simulink model "example_2"  (R2022b)
settings: Solver=VariableStepAuto  StartTime=0.0  StopTime=1  RelTol=1e-3
InitFcn:
  | %% Bộ biến đổi điện tử công suất
  | kb = 1;     % Hệ số khuếch đại khâu 1
  | f_switch = 53600; % (Hz) Tần số đóng cắt của bộ biến đổi
  | tb = 1/(2 * f_switch);   % Hằng số thời gian khâu 1
  | %% Động cơ
  | R = 0.6; % (Ohm) Điện trở động cơ
  | L = 1.5e-3; % (H) Điện cảm động cơ
  | k = 1/R; % Gain hàm truyền Plant
  | t = L/R; % Hằng số thời gian Plant
  | TL = 0.27; % Momen tải
  | ke = 0.064; % hằng số momen và hằng số sức điện động
  | J = 750e-3 * 10^(-4); % Momen quán tính động cơ
  | B = 0;
  | 
  | %% Bộ điều khiển
  | %omega_BW = 2 * pi * 1000;
  | omega_BW = 2*pi*f_switch/10;
  | Ti = t;
  | kp = R*Ti*omega_BW*sqrt(1 + (omega_BW*tb)^2)/kb;
  | ki = kp/Ti;
  | %Ts = 1e-5; % Thời gian trích mẫu
  | Ts = 1/53600;
  | % Feedforward
  | wn = 5* omega_BW;
  | %wn = 2*pi*f_switch/10; % Băng thông bộ lọc thông thấp Butterworth bậc 2
settings Model: Creator=hoang  LastModifiedBy=hoang
settings DataIOCC: ReturnWorkspaceOutputs=off

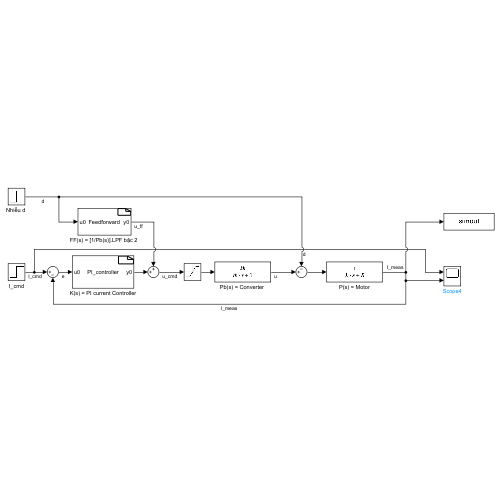
[thumbnail: Simulink's stored preview of the top-level diagram]
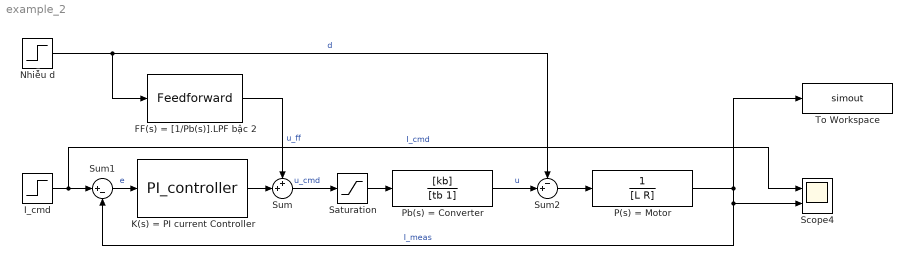
== system example_2 ==
  "FF(s) = [1/Pb(s)].LPF bậc 2 " : S-Function  FunctionName=Feedforward  Parameters=Ts,wn ,tb,kb  SFunctionModules=Feedforward_wrapper.c  SFunctionDeploymentMode=off  EnableBusSupport=off  mask(S-Function Builder){}
      mask help: Simulink:masks:SFunctionBuilder_MD
      mask init:
      | val = [[.9  0.75 0.75 1 1 .9 .9 1]',[1 1 0.75 0.75 .9 .9 1 .9]'];try , sys = get_param(gcb,'SfunBuilderFcnName');if isempty(sys), sys = get_param(gcb,'FunctionName'); end,catch, sys = get_param(gcb,'FunctionName'); end
      settings: CopyFcn=set_param(gcbh,'LinkStatus','none')  OpenFcn=sfunctionwizard(gcbh)
      mask Display:
      | plot(val(:,1),val(:,2))
      | disp(sys)
      | port_label('input',1,'u0')
      | port_label('output',1,'y0')
  I_cmd : Step  Time=0.5  SampleTime=0
  K(s) = PI current Controller : S-Function  FunctionName=PI_controller  Parameters=ki,kp,Ts  SFunctionModules=PI_controller_wrapper.c  SFunctionDeploymentMode=off  EnableBusSupport=off  mask(S-Function Builder){}
      mask help: Simulink:masks:SFunctionBuilder_MD
      mask init: same as example_2/FF(s) = [1/Pb(s)].LPF bậc 2 
      settings: CopyFcn=set_param(gcbh,'LinkStatus','none')  OpenFcn=sfunctionwizard(gcbh)
      mask Display:
      | plot(val(:,1),val(:,2))
      | disp(sys)
      | port_label('input',1,'u0')
      | port_label('output',1,'y0')
  "Nhiễu d " : Step  Time=0.5  After=40  SampleTime=0
  P(s) = Motor : TransferFcn  Denominator=[L R]
  "Pb(s) = Converter " : TransferFcn  Numerator=[kb]  Denominator=[tb 1]
  Saturation : Saturate  UpperLimit=inf  LowerLimit=-inf
  Scope4 : Scope  NumInputPorts=2
  Sum : Sum  Inputs=++|
  Sum1 : Sum  Inputs=|+-
  Sum2 : Sum  Inputs=-+|
  To Workspace : ToWorkspace  VariableName=simout  SaveFormat=Timeseries  SampleTime=-1
  wires:
  P(s) = Motor/1 -> Scope4/2, Sum1/2, To Workspace/1  "I_meas"
  Sum1/1 -> K(s) = PI current Controller/1  "e"
  K(s) = PI current Controller/1 -> Sum/2
  "Pb(s) = Converter "/1 -> Sum2/2  "u"
  Sum2/1 -> P(s) = Motor/1
  I_cmd/1 -> Scope4/1, Sum1/1  "I_cmd"
  Sum/1 -> Saturation/1  "u_cmd"
  Saturation/1 -> "Pb(s) = Converter "/1
  "Nhiễu d "/1 -> Sum2/1, "FF(s) = [1/Pb(s)].LPF bậc 2 "/1  "d"
  "FF(s) = [1/Pb(s)].LPF bậc 2 "/1 -> Sum/1  "u_ff"
